simulink model "sota_bms_aco_ekf"  (R2024b)
settings: Solver=FixedStepDiscrete  StartTime=0.0  StopTime=NASA_StopTime  FixedStep=1  RelTol=1e-3
InitFcn:
  | bms_setup('nasa')
values from neighbouring files (symbols this model uses):
  NASA_Q : value not decoded    [bms_data.sldd]
  NASA_R = 0.009881778    [bms_data.sldd]
undefined symbols (not defined in the file or in its folder): NASA_CapRatio, NASA_SOC_Guess
settings Model: DataDictionary=bms_data.sldd  Creator=sande  LastModifiedBy=sande
settings DataIOCC: SaveOutput=off
settings DebuggingCC: SignalInfNanChecking=error  AlgebraicLoopMsg=error  ArtificialAlgebraicLoopMsg=error  UnconnectedInputMsg=error  UnconnectedOutputMsg=error  UnconnectedLineMsg=error  BusObjectLabelMismatch=error  StrictBusMsg=ErrorOnBusTreatedAsVector
settings HardwareCC: ProdBitPerPointer=32  ProdBitPerSizeT=32  ProdBitPerPtrDiffT=32  ProdLargestAtomicInteger=Long  ProdLargestAtomicFloat=Double  ProdWordSize=32  ProdHWDeviceType=ARM Compatible->ARM Cortex

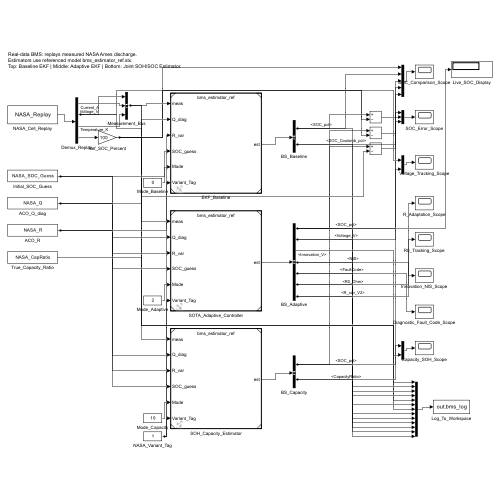
[thumbnail: Simulink's stored preview of the top-level diagram]
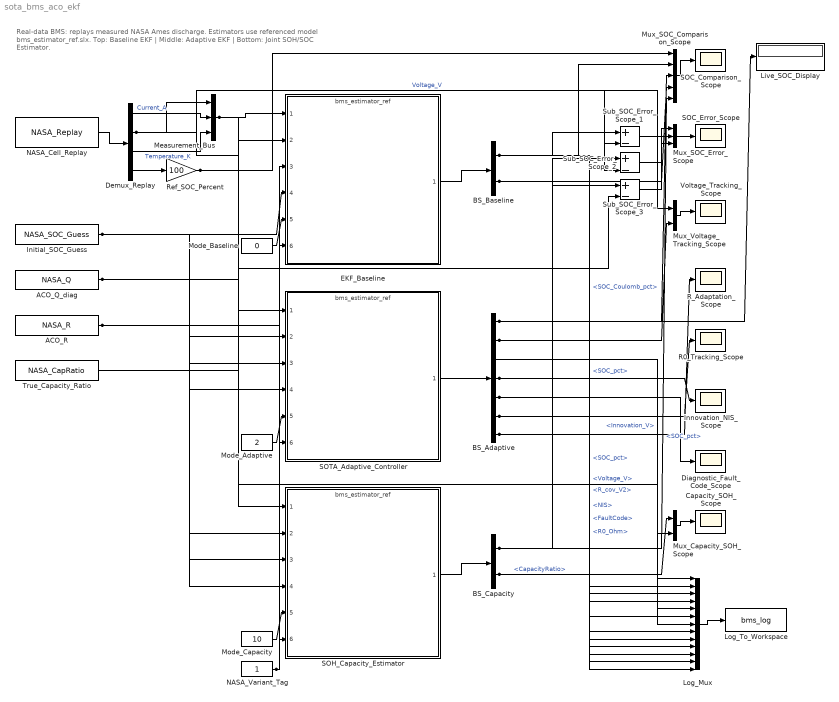
== system sota_bms_aco_ekf ==
  note: Real-data BMS: replays measured NASA Ames discharge.
      | Estimators use referenced model bms_estimator_ref.slx.
      | Top: Baseline EKF | Middle: Adaptive EKF | Bottom: Joint SOH/SOC Estimator.
  ACO_Q_diag : Constant  Value=NASA_Q  SampleTime=-1
  ACO_R : Constant  Value=NASA_R  SampleTime=-1
  BS_Adaptive : BusSelector  OutputSignals=SOC_pct,Voltage_V,Innovation_V,NIS,FaultCode,R0_Ohm,R_cov_V2
  BS_Baseline : BusSelector  OutputSignals=SOC_pct,SOC_Coulomb_pct
  BS_Capacity : BusSelector  OutputSignals=SOC_pct,CapacityRatio
  Capacity_SOH_Scope : Scope
      settings: Description=Estimated capacity ratio (SOH) | true capacity ratio
  Demux_Replay : Demux
  Diagnostic_Fault_Code_Scope : Scope
      settings: Description=Diagnostic bit-mask
  EKF_Baseline : ModelReference  ModelNameDialog=bms_estimator_ref  SimulationMode=Normal  ModelReferenceVersion=1.2
  Initial_SOC_Guess : Constant  Value=NASA_SOC_Guess  SampleTime=-1
  Innovation_NIS_Scope : Scope
      settings: Description=NIS (expect ~1)
  Live_SOC_Display : Display
  Log_Mux : Mux  Inputs=13
  Log_To_Workspace : ToWorkspace  VariableName=bms_log  SampleTime=-1
  Measurement_Bus : BusCreator  Inputs=3  OutDataTypeStr=Bus: BMS_Measurement
  Mode_Adaptive : Constant  Value=2  SampleTime=-1
  Mode_Baseline : Constant  Value=0  SampleTime=-1
  Mode_Capacity : Constant  Value=10  SampleTime=-1
  Mux_Capacity_SOH_Scope : Mux  Inputs=2
  Mux_SOC_Comparison_Scope : Mux  Inputs=5
  Mux_SOC_Error_Scope : Mux  Inputs=3
  Mux_Voltage_Tracking_Scope : Mux  Inputs=2
  NASA_Cell_Replay : FromWorkspace  VariableName=NASA_Replay  SampleTime=1  Interpolate=off  OutputAfterFinalValue=Holding final value
  NASA_Variant_Tag : Constant  SampleTime=-1
  R0_Tracking_Scope : Scope
      settings: Description=R0 used by adaptive model [ohm]
  R_Adaptation_Scope : Scope
      settings: Description=Sage-Husa measurement-noise variance R
  Ref_SOC_Percent : Gain  Gain=100
  SOC_Comparison_Scope : Scope
      settings: Description=Reference SOC | EKF | Adaptive EKF | Coulomb counting | EKF+capacity state
  SOC_Error_Scope : Scope
      settings: Description="EKF error | Adaptive EKF error | EKF+capacity error  [%]"
  SOH_Capacity_Estimator : ModelReference  ModelNameDialog=bms_estimator_ref  SimulationMode=Normal  ModelReferenceVersion=1.2
  SOTA_Adaptive_Controller : ModelReference  ModelNameDialog=bms_estimator_ref  SimulationMode=Normal  ModelReferenceVersion=1.2
  Sub_SOC_Error_Scope_1 : Sum  Inputs=+-
  Sub_SOC_Error_Scope_2 : Sum  Inputs=+-
  Sub_SOC_Error_Scope_3 : Sum  Inputs=+-
  True_Capacity_Ratio : Constant  Value=NASA_CapRatio  SampleTime=-1
  Voltage_Tracking_Scope : Scope
      settings: Description=Measured V (real cell) | Adaptive EKF predicted V
  wires:
  NASA_Cell_Replay/1 -> Demux_Replay/1
  Demux_Replay/4 -> Ref_SOC_Percent/1
  Demux_Replay/2 -> Measurement_Bus/1, Mux_Voltage_Tracking_Scope/1, Log_Mux/5  "Voltage_V"
  Demux_Replay/1 -> Measurement_Bus/2  "Current_A"
  Demux_Replay/3 -> Measurement_Bus/3  "Temperature_K"
  Measurement_Bus/1 -> EKF_Baseline/1, SOTA_Adaptive_Controller/1, SOH_Capacity_Estimator/1
  ACO_Q_diag/1 -> EKF_Baseline/2, SOTA_Adaptive_Controller/2, SOH_Capacity_Estimator/2
  ACO_R/1 -> EKF_Baseline/3, SOTA_Adaptive_Controller/3, SOH_Capacity_Estimator/3
  Initial_SOC_Guess/1 -> EKF_Baseline/4, SOTA_Adaptive_Controller/4, SOH_Capacity_Estimator/4
  NASA_Variant_Tag/1 -> EKF_Baseline/6, SOTA_Adaptive_Controller/6, SOH_Capacity_Estimator/6
  Mode_Baseline/1 -> EKF_Baseline/5
  Mode_Adaptive/1 -> SOTA_Adaptive_Controller/5
  Mode_Capacity/1 -> SOH_Capacity_Estimator/5
  EKF_Baseline/1 -> BS_Baseline/1
  SOTA_Adaptive_Controller/1 -> BS_Adaptive/1
  SOH_Capacity_Estimator/1 -> BS_Capacity/1
  Ref_SOC_Percent/1 -> Mux_SOC_Comparison_Scope/1, Sub_SOC_Error_Scope_1/2, Sub_SOC_Error_Scope_2/2, Sub_SOC_Error_Scope_3/2, Log_Mux/1
  BS_Baseline/1 -> Mux_SOC_Comparison_Scope/2, Sub_SOC_Error_Scope_1/1, Log_Mux/2  "<SOC_pct>"
  BS_Adaptive/1 -> Mux_SOC_Comparison_Scope/3, Sub_SOC_Error_Scope_2/1, Live_SOC_Display/1, Log_Mux/3  "<SOC_pct>"
  BS_Baseline/2 -> Mux_SOC_Comparison_Scope/4, Log_Mux/4  "<SOC_Coulomb_pct>"
  BS_Capacity/1 -> Mux_SOC_Comparison_Scope/5, Sub_SOC_Error_Scope_3/1, Log_Mux/12  "<SOC_pct>"
  Mux_SOC_Comparison_Scope/1 -> SOC_Comparison_Scope/1
  Sub_SOC_Error_Scope_1/1 -> Mux_SOC_Error_Scope/1
  Sub_SOC_Error_Scope_2/1 -> Mux_SOC_Error_Scope/2
  Sub_SOC_Error_Scope_3/1 -> Mux_SOC_Error_Scope/3
  Mux_SOC_Error_Scope/1 -> SOC_Error_Scope/1
  BS_Adaptive/2 -> Mux_Voltage_Tracking_Scope/2, Log_Mux/6  "<Voltage_V>"
  Mux_Voltage_Tracking_Scope/1 -> Voltage_Tracking_Scope/1
  BS_Adaptive/7 -> R_Adaptation_Scope/1, Log_Mux/11  "<R_cov_V2>"
  BS_Adaptive/6 -> R0_Tracking_Scope/1, Log_Mux/10  "<R0_Ohm>"
  BS_Adaptive/4 -> Innovation_NIS_Scope/1, Log_Mux/8  "<NIS>"
  BS_Adaptive/5 -> Diagnostic_Fault_Code_Scope/1, Log_Mux/9  "<FaultCode>"
  BS_Capacity/2 -> Mux_Capacity_SOH_Scope/1, Log_Mux/13  "<CapacityRatio>"
  True_Capacity_Ratio/1 -> Mux_Capacity_SOH_Scope/2
  Mux_Capacity_SOH_Scope/1 -> Capacity_SOH_Scope/1
  BS_Adaptive/3 -> Log_Mux/7  "<Innovation_V>"
  Log_Mux/1 -> Log_To_Workspace/1
